simulink model "commande_vectorielle_FOC"  (R2025b)
settings: Solver=ode45  StartTime=0.0  StopTime=0.1  RelTol=1e-5
undefined symbols (not defined in the file): B, J, Ki, Kp, Ld, Lq, p, psi_f, Rs, Vmax
libraries: slpidlib x2
settings Model: Creator=conte  LastModifiedBy=conte

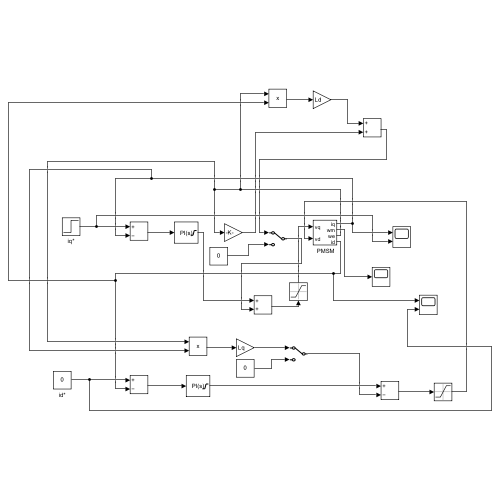
[thumbnail: Simulink's stored preview of the top-level diagram]
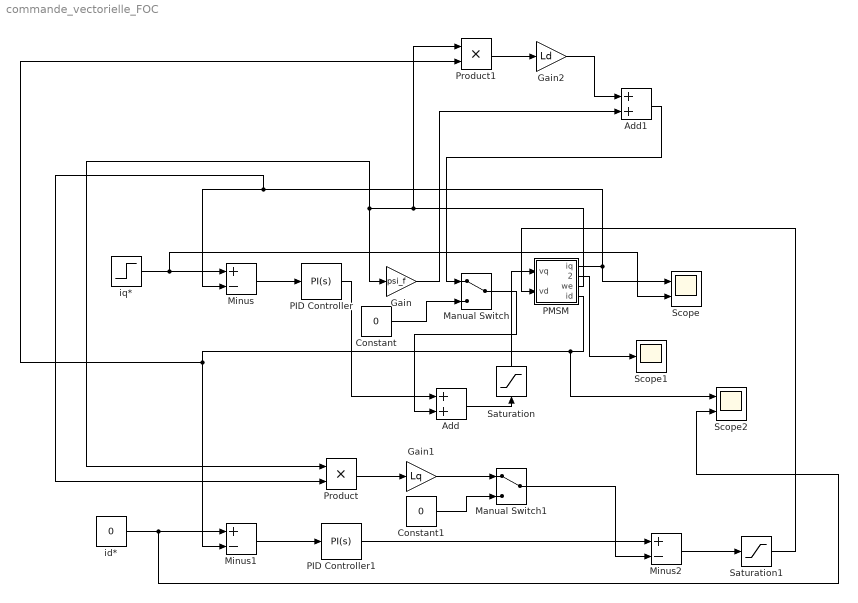
== system commande_vectorielle_FOC ==
  " PMSM" : Subsystem
  Add : Sum
  Add1 : Sum
  Constant : Constant  Value=0
  Constant1 : Constant  Value=0
  Gain : Gain  Gain=psi_f
  Gain1 : Gain  Gain=Lq
  Gain2 : Gain  Gain=Ld
  Manual Switch : ManualSwitch
  Manual Switch1 : ManualSwitch
  Minus : Sum  Inputs=+-
  Minus1 : Sum  Inputs=+-
  Minus2 : Sum  Inputs=+-
  PID Controller : slpidlib/PID Controller  Controller=PI  Form=Parallel  TimeDomain=Continuous-time  UseExternalTs=off  SampleTime=-1  IntegratorMethod=Forward Euler  FilterMethod=Forward Euler  ControllerParametersSource=internal  P=Kp  I=Ki  UseKiTs=off  D=0  UseExternalDerivativeSource=off  N=100  UseFilter=on  TunerSelectOption=Transfer Function Based (PID Tuner App)  InitialConditionSource=internal  InitialConditionForIntegrator=0  InitialConditionForFilter=0  DifferentiatorICPrevScaledInput=0  ExternalReset=none  TrackingMode=off  Kt=1  LimitOutput=on  SatLimitsSource=internal  UpperSaturationLimit=Vmax  LowerSaturationLimit=-Vmax  LinearizeAsGain=on  AntiWindupMode=clamping  Kb=1  LimitIntegrator=on  UpperIntegratorSaturationLimit=Vmax  LowerIntegratorSaturationLimit=-Vmax  POutMin=[]  POutMax=[]  IOutMin=[]  IOutMax=[]  DOutMin=[]  DOutMax=[]  NOutMin=[]  NOutMax=[]  SumOutMin=[]  SumOutMax=[]  SaturationOutMin=[]  SaturationOutMax=[]  PParamMin=[]  PParamMax=[]  IParamMin=[]  IParamMax=[]  DParamMin=[]  DParamMax=[]  NParamMin=[]  NParamMax=[]  KbParamMin=[]  KbParamMax=[]  KtParamMin=[]  KtParamMax=[]  KbOutMin=[]  KbOutMax=[]  KtOutMin=[]  KtOutMax=[]  IntegratorOutMin=[]  IntegratorOutMax=[]  FilterOutMin=[]  FilterOutMax=[]  SumI1OutMin=[]  SumI1OutMax=[]  SumI2OutMin=[]  SumI2OutMax=[]  SumI3OutMin=[]  SumI3OutMax=[]  SumI4OutMin=[]  SumI4OutMax=[]  SumDOutMin=[]  SumDOutMax=[]  DifferentiatorOutMin=[]  DifferentiatorOutMax=[]  FilterDiffOutCoefMin=[]  FilterDiffOutCoefMax=[]  ReciprocalOutMin=[]  ReciprocalOutMax=[]  SumDenOutMin=[]  SumDenOutMax=[]  SumNumOutMin=[]  SumNumOutMax=[]  DivideOutMin=[]  DivideOutMax=[]  UdiffTsProdOutMin=[]  UdiffTsProdOutMax=[]  NTsProdOutMin=[]  NTsProdOutMax=[]  UintegralTsProdOutMin=[]  UintegralTsProdOutMax=[]  UngainTsProdOutMin=[]  UngainTsProdOutMax=[]  ClampingZeroOutDataTypeStr=Inherit: Inherit via back propagation  ClampingZeroOutMin=[]  ClampingZeroOutMax=[]  FilterDenConstantOutDataTypeStr=Inherit: Inherit via back propagation  FilterDenConstantOutMin=[]  FilterDenConstantOutMax=[]  PCopyOutDataTypeStr=Inherit: Inherit via back propagation  PCopyOutMin=[]  PCopyOutMax=[]  NCopyOutDataTypeStr=Inherit: Inherit via back propagation  NCopyOutMin=[]  NCopyOutMax=[]  IntegratorContinuousStateAttributes=''  IntegratorStateMustResolveToSignalObject=off  IntegratorRTWStateStorageClass=Auto  FilterContinuousStateAttributes=''  FilterStateMustResolveToSignalObject=off  FilterRTWStateStorageClass=Auto  ParallelPVariant=InternalParameters  IdealPVariant=Disabled  IVariant=InternalParameters  DVariant=Disabled  IntegratorVariant=Continuous  SatVariant=Enabled  AWVariant=ContClampingParallel  PCopyVariant=Disabled  TRVariant=Disabled  FdbkBlocksVariant=Forward  IdealPFdbkVariant=Disabled  SatFdbkVariant=Disabled  DerivativeFilterVariant=Disabled  NVariant=Disabled  NCopyVariant=Disabled_SignalSpec  FilterICVariant=Disabled  IntegratorICVariant=InternalICs  ExternalResetVariant=Disabled  TRSumVariant=Passthrough  SumFdbkVariant=Disabled  SumVariant=Sum_PI  TsampFilterVariant=InternalTs  TsampNgainVariant=Passthrough  TsampIntegralVariant=Disabled_SignalSpec  ExternalSaturationOutDataTypeStr=Inherit: Same as second input  DerivativeSourceVariant=Disabled  PreIntVariant=InternalPreInt
  PID Controller1 : slpidlib/PID Controller  Controller=PI  Form=Parallel  TimeDomain=Continuous-time  UseExternalTs=off  SampleTime=-1  IntegratorMethod=Forward Euler  FilterMethod=Forward Euler  ControllerParametersSource=internal  P=Kp  I=Ki  UseKiTs=off  D=0  UseExternalDerivativeSource=off  N=100  UseFilter=on  TunerSelectOption=Transfer Function Based (PID Tuner App)  InitialConditionSource=internal  InitialConditionForIntegrator=0  InitialConditionForFilter=0  DifferentiatorICPrevScaledInput=0  ExternalReset=none  TrackingMode=off  Kt=1  LimitOutput=on  SatLimitsSource=internal  UpperSaturationLimit=Vmax  LowerSaturationLimit=-Vmax  LinearizeAsGain=on  AntiWindupMode=clamping  Kb=1  LimitIntegrator=on  UpperIntegratorSaturationLimit=Vmax  LowerIntegratorSaturationLimit=-Vmax  POutMin=[]  POutMax=[]  IOutMin=[]  IOutMax=[]  DOutMin=[]  DOutMax=[]  NOutMin=[]  NOutMax=[]  SumOutMin=[]  SumOutMax=[]  SaturationOutMin=[]  SaturationOutMax=[]  PParamMin=[]  PParamMax=[]  IParamMin=[]  IParamMax=[]  DParamMin=[]  DParamMax=[]  NParamMin=[]  NParamMax=[]  KbParamMin=[]  KbParamMax=[]  KtParamMin=[]  KtParamMax=[]  KbOutMin=[]  KbOutMax=[]  KtOutMin=[]  KtOutMax=[]  IntegratorOutMin=[]  IntegratorOutMax=[]  FilterOutMin=[]  FilterOutMax=[]  SumI1OutMin=[]  SumI1OutMax=[]  SumI2OutMin=[]  SumI2OutMax=[]  SumI3OutMin=[]  SumI3OutMax=[]  SumI4OutMin=[]  SumI4OutMax=[]  SumDOutMin=[]  SumDOutMax=[]  DifferentiatorOutMin=[]  DifferentiatorOutMax=[]  FilterDiffOutCoefMin=[]  FilterDiffOutCoefMax=[]  ReciprocalOutMin=[]  ReciprocalOutMax=[]  SumDenOutMin=[]  SumDenOutMax=[]  SumNumOutMin=[]  SumNumOutMax=[]  DivideOutMin=[]  DivideOutMax=[]  UdiffTsProdOutMin=[]  UdiffTsProdOutMax=[]  NTsProdOutMin=[]  NTsProdOutMax=[]  UintegralTsProdOutMin=[]  UintegralTsProdOutMax=[]  UngainTsProdOutMin=[]  UngainTsProdOutMax=[]  ClampingZeroOutDataTypeStr=Inherit: Inherit via back propagation  ClampingZeroOutMin=[]  ClampingZeroOutMax=[]  FilterDenConstantOutDataTypeStr=Inherit: Inherit via back propagation  FilterDenConstantOutMin=[]  FilterDenConstantOutMax=[]  PCopyOutDataTypeStr=Inherit: Inherit via back propagation  PCopyOutMin=[]  PCopyOutMax=[]  NCopyOutDataTypeStr=Inherit: Inherit via back propagation  NCopyOutMin=[]  NCopyOutMax=[]  IntegratorContinuousStateAttributes=''  IntegratorStateMustResolveToSignalObject=off  IntegratorRTWStateStorageClass=Auto  FilterContinuousStateAttributes=''  FilterStateMustResolveToSignalObject=off  FilterRTWStateStorageClass=Auto  ParallelPVariant=InternalParameters  IdealPVariant=Disabled  IVariant=InternalParameters  DVariant=Disabled  IntegratorVariant=Continuous  SatVariant=Enabled  AWVariant=ContClampingParallel  PCopyVariant=Disabled  TRVariant=Disabled  FdbkBlocksVariant=Forward  IdealPFdbkVariant=Disabled  SatFdbkVariant=Disabled  DerivativeFilterVariant=Disabled  NVariant=Disabled  NCopyVariant=Disabled_SignalSpec  FilterICVariant=Disabled  IntegratorICVariant=InternalICs  ExternalResetVariant=Disabled  TRSumVariant=Passthrough  SumFdbkVariant=Disabled  SumVariant=Sum_PI  TsampFilterVariant=InternalTs  TsampNgainVariant=Passthrough  TsampIntegralVariant=Disabled_SignalSpec  ExternalSaturationOutDataTypeStr=Inherit: Same as second input  DerivativeSourceVariant=Disabled  PreIntVariant=InternalPreInt
  Product : Product
  Product1 : Product
  Saturation : Saturate  UpperLimit=Vmax  LowerLimit=-Vmax
  Saturation1 : Saturate  UpperLimit=Vmax  LowerLimit=-Vmax
  Scope : Scope  NumInputPorts=2
      settings: ActiveDisplayYMinimum=-0.24999999999999994  ActiveDisplayYMaximum=2.25
  Scope1 : Scope
      settings: ActiveDisplayYMinimum=-44.0462383231296  ActiveDisplayYMaximum=396.41614490816647
  Scope2 : Scope  NumInputPorts=2
      settings: ActiveDisplayYMinimum=-1  ActiveDisplayYMaximum=1  DataLoggingVariableName=ScopeData2
  id* : Constant  Value=0
  iq* : Step  Time=0.001  After=2  SampleTime=0
  wires:
  " PMSM"/1(iq) -> Minus/2, Product/2, Scope/1
  iq*/1 -> Minus/1, Scope/2
  Minus/1 -> PID Controller/1
  " PMSM"/3(we) -> Product1/1, Gain/1, Product/1
  Constant/1 -> Manual Switch/2
  PID Controller/1 -> Add/1
  Manual Switch/1 -> Add/2
  Add/1 -> Saturation/1
  " PMSM"/2(wm) -> Scope1/1
  Saturation/1 -> " PMSM"/1(vq)
  id*/1 -> Scope2/2, Minus1/1
  " PMSM"/4(id) -> Scope2/1, Minus1/2, Product1/2
  Minus1/1 -> PID Controller1/1
  Product/1 -> Gain1/1
  Gain1/1 -> Manual Switch1/1
  Constant1/1 -> Manual Switch1/2
  PID Controller1/1 -> Minus2/1
  Manual Switch1/1 -> Minus2/2
  Minus2/1 -> Saturation1/1
  Saturation1/1 -> " PMSM"/2(vd)
  Gain/1 -> Add1/2
  Add1/1 -> Manual Switch/1
  Product1/1 -> Gain2/1
  Gain2/1 -> Add1/1

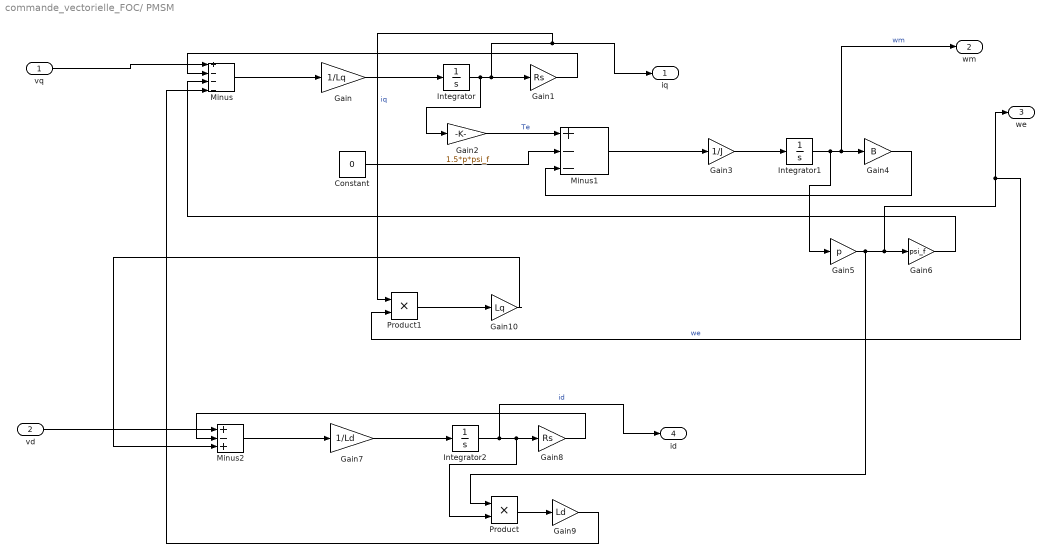
== system commande_vectorielle_FOC/ PMSM ==
  vq : Inport
  vd : Inport  Port=2
  Constant : Constant  Value=0
  Gain : Gain  Gain=1/Lq
  Gain1 : Gain  Gain=Rs
  Gain10 : Gain  Gain=Lq
  Gain2 : Gain  Gain=1.5*p*psi_f
  Gain3 : Gain  Gain=1/J
  Gain4 : Gain  Gain=B
  Gain5 : Gain  Gain=p
  Gain6 : Gain  Gain=psi_f
  Gain7 : Gain  Gain=1/Ld
  Gain8 : Gain  Gain=Rs
  Gain9 : Gain  Gain=Ld
  Integrator : Integrator
  Integrator1 : Integrator
  Integrator2 : Integrator
  Minus : Sum  Inputs=+---
  Minus1 : Sum  Inputs=+--
  Minus2 : Sum  Inputs=+-+
  Product : Product
  Product1 : Product
  iq : Outport
  wm : Outport  Port=2
  we : Outport  Port=3
  id : Outport  Port=4
  wires:
  vq/1 -> Minus/1
  Minus/1 -> Gain/1
  Integrator/1 -> Gain2/1, iq/1, Product1/1, Gain1/1  "iq"
  Gain1/1 -> Minus/2
  Gain/1 -> Integrator/1
  Gain2/1 -> Minus1/1  "Te"
  Constant/1 -> Minus1/2
  Minus1/1 -> Gain3/1
  Gain3/1 -> Integrator1/1
  Integrator1/1 -> Gain5/1, wm/1, Gain4/1  "wm"
  Gain4/1 -> Minus1/3
  Gain5/1 -> Product/1, Gain6/1, Product1/2, we/1  "we"
  Gain6/1 -> Minus/3
  Gain8/1 -> Minus2/2
  Gain7/1 -> Integrator2/1
  Minus2/1 -> Gain7/1
  Integrator2/1 -> id/1, Product/2, Gain8/1  "id"
  vd/1 -> Minus2/1
  Product/1 -> Gain9/1
  Gain9/1 -> Minus/4
  Product1/1 -> Gain10/1
  Gain10/1 -> Minus2/3
